simulink model "DTC_step625_20261016_164342_084"  (R2025b)
settings: Solver=FixedStepDiscrete  StartTime=0  StopTime=3.5  FixedStep=6.2500000000000005e-07  MaxStep=1e-3  RelTol=1e-3  EnableMultiTasking=on
model workspace (MAT data in the model file):
  F = 0.0106
  H = 0.2734
  IphasePeak = 243.46443504
  J_kgm2 = 2.52388816871
  Ki_wr = 3134.2
  Kp_wr = 65.47
  Llr_H = 0.000328787586604
  Llr_pu = 0.067199338843
  Lls_H = 0.000328787586604
  Lm_H = 0.0132934166218
  Lm_pu = 2.7169785124
  Pn = 164000
  Rr_pu = 0.0112002512397
  Rrr = 0.020659
  Rss = 0.025639
  Tbase = 870.047022236
  Ts = 6.25e-07
  Tsc = 5e-05
  Vdc = 750
  Vn = 550
  VphasePeak = 449.07311951
  Xlr = 0.12395
  Xls = 0.12395
  Xm = 5.0115
  Zbase = 1.84451219512
  fn = 60
  fswFOC = 5000
  imRef_pu = 0.36805591043
  omegaBase = 188.495559215
  p = 2
  psin = 1.19120344633
  rpmBase = 1800
undefined symbols (not defined in the file): ee
libraries: nesl_utility x12, ee_lib x10, fl_lib x5, eeAsmDirectTorqueControl x1, slpidlib x1
Description:
  | Asynchronous Machine Direct Torque Control
settings Model: Creator=The MathWorks, Inc.  LastModifiedBy=Ulterior Engineering
settings SolverCC: AlgebraicLoopSolver=TrustRegion  AutoInsertRateTranBlk=on  MaxZcPerStep=1.0
settings DataIOCC: MaxDataPoints=510000  SaveOperatingPoint=on  SaveFormat=StructureWithTime  SaveOutput=off  SignalLogging=off  SignalLoggingName=logsout_InductionMachineDTC
settings OptimizationCC: ReuseModelBlockBuffer=off  ExpressionDepthLimit=2147483647.0  LifeSpan=inf
settings DebuggingCC: AlgebraicLoopMsg=error  SolverPrmCheckMsg=warning  MultiTaskRateTransMsg=warning  UnconnectedInputMsg=warning  UnconnectedOutputMsg=warning  UnconnectedLineMsg=warning  StateNameClashWarn=warning  SFUnexpectedBacktrackingDiag=warning  SFNoUnconditionalDefaultTransitionDiag=warning  SFExecutionAtInitializationDiag=none  ArithmeticOperatorsInVariantConditions=warning
settings HardwareCC: ProdBitPerPointer=32.0  ProdBitPerSizeT=32.0  ProdBitPerPtrDiffT=32.0  ProdLargestAtomicFloat=None  ProdIntDivRoundTo=Undefined  ProdEndianess=Unspecified  ProdWordSize=32.0  ProdHWDeviceType=32-bit Generic
settings ModelReferenceCC: EnableRefExpFcnMdlSchedulingChecks=on  PropagateSignalLabelsOutOfModel=off
settings SFSimCC: SimUseLocalCustomCode=off  CustomCodeUndefinedFunction=UseInterfaceOnly
settings RTWCC: RTWUseLocalCustomCode=off  GPUComputeCapability=3.5  DLArmComputeVersion=19.05
settings CodeAppCC: StateflowObjectComments=on
settings GRTTargetCC: TargetLangStandard=C89/C90 (ANSI)
settings ConfigComp: CovMetricSettings=dw  CovSaveCumulativeToWorkspaceVar=on  CovSaveSingleToWorkspaceVar=on  CovExternalEMLEnable=off  CovSFcnEnable=off
settings SimscapeCC: SimscapeLogSimulationStatistics=on  SimscapeLogName=simlog_InductionMachineDTC  SimscapeLogDecimation=5.0  SimscapeLogDataHistory=510000.0

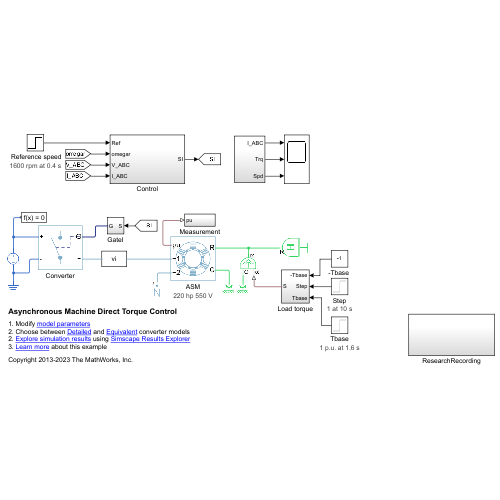
[thumbnail: Simulink's stored preview of the top-level diagram]
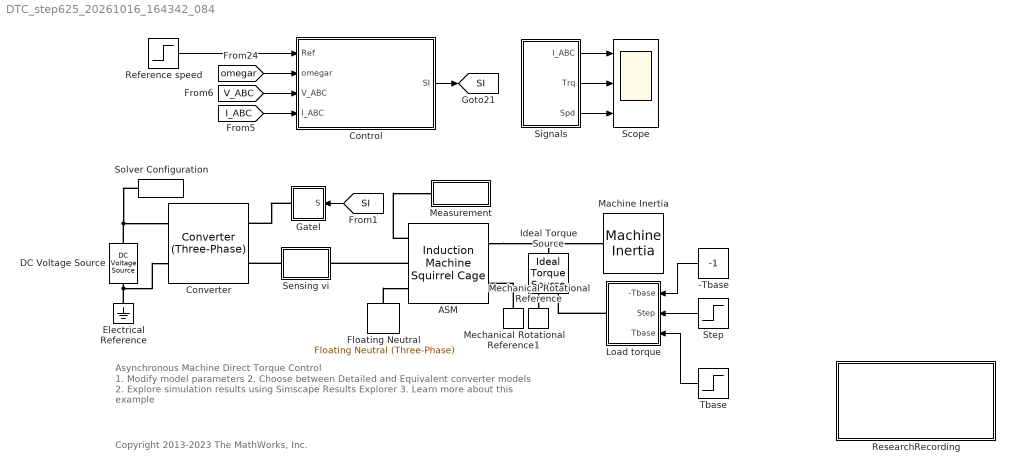
== system DTC_step625_20261016_164342_084 ==
  note: Asynchronous Machine Direct Torque Control
  note: 1. Modify model parameters
      | 2. Choose between Detailed and Equivalent converter models
      | 2. Explore simulation results using Simscape Results Explorer
      | 3. Learn more about this example
  note: Copyright 2013-2023 The MathWorks, Inc.
  " Reference speed" : Step  Time=0.4  After=1600  SampleTime=Tsc
      settings: AttributesFormatString=%<After> rpm at %<Time> s
  "-Tbase " : Constant  Value=-1  SampleTime=Ts
  ASM : ee_lib/Electromechanical/Asynchronous/Induction Machine Squirrel Cage  port_option=ee.enum.threePhasePort.composite  SRated=Pn V*A  VRated=Vn V  FRated=fn Hz  nPolePairs=p  param_unit=ee.enum.unit.si  squirrel_cage=ee.enum.squirrelcage.Single  zero_sequence=ee.enum.park.zerosequence.include  initialization_option=ee.enum.asm.initialization.fluxvariables  Rs=Rss Ohm  Xls=Xls Ohm  pu_Rs=0.0258  pu_Lls=0.0413  Rrd=0.020659 Ohm  Xlrd=Xlr Ohm  pu_Rrd=0.0145  pu_Llrd=0.0424  Rrd1=0.28 Ohm  Xlrd1=0.82 Ohm  Rrd2=0.28 Ohm  Xlrd2=0.82 Ohm  pu_Rrd1=0.0290  pu_Llrd1=0.0848  pu_Rrd2=0.0290  pu_Llrd2=0.0848  Xm=Xm Ohm  pu_Lm=1.7562  X0=Xls Ohm  pu_L0=0.0413  saturation_option=0  saturation_i=[0, 4, 9, 18, 25, 34, 50, 68, 95, 120] A  saturation_v=[0, 88, 154, 198, 220, 242, 264, 286, 308, 330] V  pu_saturation_i=[0, .176, .396, .792, 1.1, 1.496, 2.2, 2.992, 4.18, 5.28]  pu_saturation_v=[0, .4, .7, .9, 1, 1.1, 1.2, 1.3, 1.4, 1.4864]  connection_option=int32(ee.enum.Connection.delta)  angular_position_specify=off  angular_position_priority=None  angular_position=0 deg  angular_position_nominal_specify=off  angular_position_nominal_value=1  angular_position_nominal_unit=deg  pu_psids_specify=off  pu_psids_priority=None  pu_psids=0  pu_psids_nominal_specify=off  pu_psids_nominal_value=1  pu_psids_nominal_unit=1  pu_psiqs_specify=off  pu_psiqs_priority=None  pu_psiqs=0  pu_psiqs_nominal_specify=off  pu_psiqs_nominal_value=1  pu_psiqs_nominal_unit=1  pu_psi0s_specify=off  pu_psi0s_priority=None  pu_psi0s=0  pu_psi0s_nominal_specify=off  pu_psi0s_nominal_value=1  pu_psi0s_nominal_unit=1  pu_psidr_specify=off  pu_psidr_priority=None  pu_psidr=0  pu_psidr_nominal_specify=off  pu_psidr_nominal_value=1  pu_psidr_nominal_unit=1  pu_psiqr_specify=off  pu_psiqr_priority=None  pu_psiqr=0  pu_psiqr_nominal_specify=off  pu_psiqr_nominal_value=1  pu_psiqr_nominal_unit=1  pu_psidr1_specify=off  pu_psidr1_priority=None  pu_psidr1=0  pu_psidr1_nominal_specify=off  pu_psidr1_nominal_value=1  pu_psidr1_nominal_unit=1  pu_psiqr1_specify=off  pu_psiqr1_priority=None  pu_psiqr1=0  pu_psiqr1_nominal_specify=off  pu_psiqr1_nominal_value=1  pu_psiqr1_nominal_unit=1  pu_psidr2_specify=off  pu_psidr2_priority=None  pu_psidr2=0  pu_psidr2_nominal_specify=off  pu_psidr2_nominal_value=1  pu_psidr2_nominal_unit=1  pu_psiqr2_specify=off  pu_psiqr2_priority=None  pu_psiqr2=0  pu_psiqr2_nominal_specify=off  pu_psiqr2_nominal_value=1  pu_psiqr2_nominal_unit=1  psids_specify=off  psids_priority=None  psids=0 Wb  psids_nominal_specify=off  psids_nominal_value=1  psids_nominal_unit=Wb  psiqs_specify=off  psiqs_priority=None  psiqs=0 Wb  psiqs_nominal_specify=off  psiqs_nominal_value=1  psiqs_nominal_unit=Wb  psi0s_specify=off  psi0s_priority=None  psi0s=0 Wb  psi0s_nominal_specify=off  psi0s_nominal_value=1  psi0s_nominal_unit=Wb  psidr_specify=off  psidr_priority=None  psidr=0 Wb  psidr_nominal_specify=off  psidr_nominal_value=1  psidr_nominal_unit=Wb  psiqr_specify=off  psiqr_priority=None  psiqr=0 Wb  psiqr_nominal_specify=off  psiqr_nominal_value=1  psiqr_nominal_unit=Wb  psidr1_specify=off  psidr1_priority=None  psidr1=0 Wb  psidr1_nominal_specify=off  psidr1_nominal_value=1  psidr1_nominal_unit=Wb  psiqr1_specify=off  psiqr1_priority=None  psiqr1=0 Wb  psiqr1_nominal_specify=off  psiqr1_nominal_value=1  psiqr1_nominal_unit=Wb  psidr2_specify=off  psidr2_priority=None  psidr2=0 Wb  psidr2_nominal_specify=off  psidr2_nominal_value=1  psidr2_nominal_unit=Wb  psiqr2_specify=off  psiqr2_priority=None  psiqr2=0 Wb  psiqr2_nominal_specify=off  psiqr2_nominal_value=1  psiqr2_nominal_unit=Wb  slip_specify=off  slip_priority=None  slip=0  slip_nominal_specify=off  slip_nominal_value=1  slip_nominal_unit=1  real_power_generated_specify=off  real_power_generated_priority=None  real_power_generated=0 W  real_power_generated_nominal_specify=off  real_power_generated_nominal_value=1  real_power_generated_nominal_unit=W  mechanical_power_consumed_specify=off  mechanical_power_consumed_priority=None  mechanical_power_consumed=0 W  mechanical_power_consumed_nominal_specify=off  mechanical_power_consumed_nominal_value=1  mechanical_power_consumed_nominal_unit=W  Tmeas=298.15 K  alpha=3.93e-3 1/K  alpha_cage=4.4e-3 1/K  stator_thermal_mass=100 J/K  rotor_thermal_mass=200 J/K  temperatureA_specify=off  temperatureA_priority=High  temperatureA=25 degC  temperatureA_nominal_specify=off  temperatureA_nominal_value=1  temperatureA_nominal_unit=degC  temperatureB_specify=off  temperatureB_priority=High  temperatureB=25 degC  temperatureB_nominal_specify=off  temperatureB_nominal_value=1  temperatureB_nominal_unit=degC  temperatureC_specify=off  temperatureC_priority=High  temperatureC=25 degC  temperatureC_nominal_specify=off  temperatureC_nominal_value=1  temperatureC_nominal_unit=degC  temperatureR_specify=off  temperatureR_priority=High  temperatureR=25 degC  temperatureR_nominal_specify=off  temperatureR_nominal_value=1  temperatureR_nominal_unit=degC
      settings: AttributesFormatString=220 hp 550 V  InternalSimscapePortConfiguration="{\"Bottom\":[],\"Left\":[{\"id\":\"R\",\"label\":\"R\",\"type\":\"foundation.mechanical.rotational.rotational\"},{\"id\":\"C\",\"label\":\"C\",\"type\":\"foundation.mechanical.rotational.rotational\"}],\"Right\":[{\"id\":\"pu_output\",\"label\":\"pu\",\"type\":\"output\"},{\"id\":\"N1\",\"label\":\"~1\",\"type\":\"foundation.electrical.three_phase\"},{\"id\":\"N2\",\"label\":\"~2\",\"type\":\"foundation.electrical.three_phase\"}],\"Top\":[]}"
  Control : Subsystem
  Converter : ee_lib/Semiconductors & Converters/Converters/Converter (Three-Phase)  port_option=ee.enum.threePhasePort.composite  fidelity_option=ee.enum.converters.fidelity.detailed  device_type=3  showThermalPort=false  K=0  Vth=0.5 V  Vgt=1 V  Vgt_off=-1 V  Ih=1 A  Vf=0.8 V  Ron=0.001 Ohm  Rds=0.001 Ohm  Goff=1e-5 1/Ohm  Eon_scalar=22.86e-3 J  Eoff_scalar=17.14e-3 J  Eoff_natural_commutation=10e-3 J  Voff=300 V  Iout_scalar=600 A  onCurrentMeasDelay=0 s  useCurrentFromPreviousCycle=false  useVoltageFromPreviousCycle=false  diode_param=2  diode_Vf=0.8 V  diode_Ron=0.001 Ohm  diode_Goff=1e-5 1/Ohm  diode_C=50 nF  diode_iRM=-235 A  diode_iF=300 A  diode_idot=-50 A/us  diode_trr_param=1  diode_trr_factor=3  diode_trr=15 us  diode_Qrr=1.5e+3 s*uA  diode_rec_loss_model=ee.enum.diode.reverseRecoveryModel.fixed  diode_ErecVal=0 J  diode_scaleWithIandV=false  diode_ErecMat=zeros(2, 3) J  diode_TjrecVec=[298.15, 398.15] K  diode_IfrecVec=[.1, 1, 10] A  diode_IrecVal=10 A  diode_VrecVal=10 V  diode_tFilter=1 / 1000 / 100 s  thermal_network_parameterization=ee.enum.thermalNetworkTopology.external  Rth=[.08, .5] K/W  Rth_Cauer=[.08, .1, .5] K/W  Rth_Foster=[.08, .14, .22, .16] K/W  thermal_mass_parameterization=ee.enum.thermalNetwork.timeconstant  thermal_mass=[.01, .5] J/K  thermal_mass_Cauer=[.01, .1, .5] J/K  thermal_mass_Foster=[.001, .005, .05, .5] J/K  thermal_time_constant=[.001, .2] s  thermal_time_constant_Cauer=[.001, .1, .2] s  thermal_time_constant_Foster=[7e-05, .0007, .01, .08] s  thermal_mass_initial_temperatures=[25, 25] degC  thermal_mass_initial_temperatures_Cauer=[25, 25, 25] degC  junction_thermal_mass=0.01 J/K  Tvec_initial_Foster=[25, 25, 25, 25] degC  snubber_type=0  Cs=1e-7 F  Rs=0.1 Ohm  Vce_loss=[0, 150, 300] V
  DC Voltage Source : fl_lib/Electrical/Electrical Sources/DC Voltage Source  v0=750 V
  Electrical Reference : fl_lib/Electrical/Electrical Elements/Electrical Reference
  Floating Neutral : ee_lib/Connectors & References/Floating Neutral (Three-Phase)  G_parasitic=1e-12 1/Ohm
      settings: InternalSimscapePortConfiguration="{\"Bottom\":[],\"Left\":[{\"id\":\"N\",\"label\":\"~\",\"type\":\"foundation.electrical.three_phase\"}],\"Right\":[],\"Top\":[]}"
  GateI : Subsystem
  Ideal Torque Source : fl_lib/Mechanical/Mechanical Sources/Ideal Torque Source
  Load torque : Subsystem
  Machine Inertia : ee_lib/Electromechanical/Mechanical/Machine Inertia  SRated=Pn V*A  FRated=fn Hz  nPolePairs=p  inertia_option=2  J=27548 kg*m^2  H=H s*W/V/A  damper_option=2  D=39.0509 N*m/(rad/s)  pu_D=F  initialization_option=2  fMechanical0=60 Hz  fElectrical0=0 Hz
      settings: InternalSimscapePortConfiguration="{\"Bottom\":[],\"Left\":[{\"id\":\"R\",\"label\":\"R\",\"type\":\"foundation.mechanical.rotational.rotational\"}],\"Right\":[],\"Top\":[]}"
  Measurement : Subsystem
  Mechanical Rotational Reference : fl_lib/Mechanical/Rotational Elements/Mechanical Rotational Reference
  Mechanical Rotational Reference1 : fl_lib/Mechanical/Rotational Elements/Mechanical Rotational Reference
  ResearchRecording : Subsystem
  Scope : Scope  NumInputPorts=3
      settings: ActiveDisplayYMinimum=-2097.68895  ActiveDisplayYMaximum=2224.93237
  Sensing vi : Subsystem
      mask Display: disp('vi')
  Signals : Subsystem
  Solver Configuration : nesl_utility/Solver Configuration  PhysicalDomain=network_engine_domain  SubClassName=solver  LeftPortType=input  RightPortType=generic  Tones=[]  Harmonics=[]  SimulateNoise=off  Profile=off  UseLocalSampling=off  EnableSwitchedLinearOptims=on  FrequencyDomain=off  UseCCode=off  RelTol=0.001  AbsTol=1e-06  MinStep=1e-09  ToWorkspace=off  RevertToSquareIcSolve=off  NumHomotopyIterations=100  PhasorMode=off  PhasorModeNumHarmonics=1  ConsistencySolver=NEWTON_FTOL  IndexReductionMethod=DerivativeReplacement  DoDC=off  ResidualTolerance=1e-09  ConsistencyTolSource=GLOBAL  ConsistencyAbsTol=0.001  ConsistencyRelTol=0.001  ConsistencyTolFactor=0.001  UseLocalSolver=on  LocalSolverChoice=NE_BACKWARD_EULER_ADVANCER  ResolveIndetEquations=on  FunctionEvalNumThread=1  LocalSolverSampleTime=6.2500000000000005e-07  DoFixedCost=on  MaxNonlinIter=10  MaxModeIter=4  ComputeImpulses=off  ImpulseIterations=2  LinearAlgebra=auto  LinearAlgebraNumThread=0  EquationFormulation=NE_TIME_EF  DelaysMemoryBudget=1024  AutomaticFiltering=on  FilteringTimeConstant=0.001  PartitionStorageMethod=AS_NEEDED  PartitionMemoryBudget=1024  PartitionMethod=ROBUST  MultibodyUseLocalSolver=off  MultibodyLocalSolverChoice=ODE1  MultibodyLocalSolverSampleTime=0.001
  Step : Step  Time=10  SampleTime=Ts
      settings: AttributesFormatString=%<After> at %<Time> s
  Tbase : Step  Time=1.6  SampleTime=Ts
      settings: AttributesFormatString=%<After> p.u. at %<Time> s
  tag scope: SI=global
  wires:
  [SI] -> GateI/1(S)
  Signals/1(I_ABC) -> Scope/1
  Signals/2(Trq) -> Scope/2
  Signals/3(Spd) -> Scope/3
  [omegar] -> Control/2(omegar)
  [V_ABC] -> Control/3(V_ABC)
  [I_ABC] -> Control/4(I_ABC)
  Control/1(SI) -> [SI]
  "-Tbase "/1 -> Load torque/1(-Tbase)
  Step/1 -> Load torque/2(Step)
  Tbase/1 -> Load torque/3(Tbase)
  " Reference speed"/1 -> Control/1(Ref)
  connections:
  DC Voltage Source/LConn1 -- Solver Configuration/RConn1 -- Converter/RConn1
  Electrical Reference/LConn1 -- Converter/RConn2 -- DC Voltage Source/RConn1
  Sensing vi/LConn1 -- Converter/LConn2
  ASM/RConn2 -- Sensing vi/RConn1
  ASM/LConn1 -- Ideal Torque Source/LConn1 -- Machine Inertia/LConn1
  Ideal Torque Source/RConn2 -- Mechanical Rotational Reference/LConn1
  GateI/RConn1 -- Converter/LConn1
  Floating Neutral/LConn1 -- ASM/RConn3
  ASM/RConn1 -- Measurement/RConn1
  Mechanical Rotational Reference1/LConn1 -- ASM/LConn2
  Load torque/RConn1 -- Ideal Torque Source/RConn1

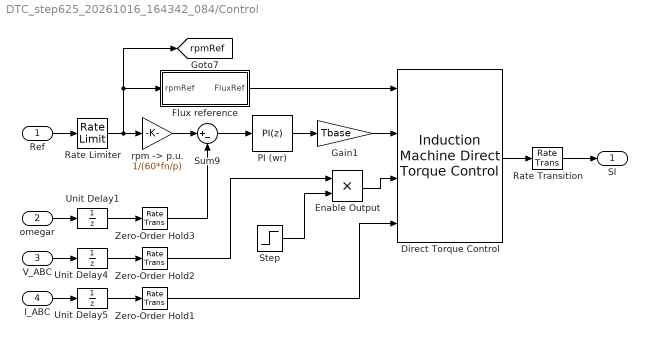
== system DTC_step625_20261016_164342_084/Control ==
  Ref : Inport
  omegar : Inport  Port=2
  V_ABC : Inport  Port=3
  I_ABC : Inport  Port=4
  " Direct Torque Control" : eeAsmDirectTorqueControl/Induction Machine Direct Torque Control  Rs=Rss  p=p  FluxHystBand=.2  THystBand=100  Ts=Tsc
  Enable Output : Product
  Flux reference : Subsystem
  Gain1 : Gain  Gain=Tbase
  PI (wr) : slpidlib/PID Controller  Controller=PI  Form=Parallel  TimeDomain=Discrete-time  UseExternalTs=off  SampleTime=Tsc  IntegratorMethod=Forward Euler  FilterMethod=Forward Euler  ControllerParametersSource=internal  P=Kp_wr  I=Ki_wr  UseKiTs=off  D=0  UseExternalDerivativeSource=off  N=100  UseFilter=on  TunerSelectOption=Transfer Function Based (PID Tuner App)  InitialConditionSource=internal  InitialConditionForIntegrator=0  InitialConditionForFilter=0  DifferentiatorICPrevScaledInput=0  ExternalReset=none  TrackingMode=off  Kt=1  LimitOutput=on  SatLimitsSource=internal  UpperSaturationLimit=2  LowerSaturationLimit=-2  LinearizeAsGain=on  AntiWindupMode=back-calculation  Kb=1000  LimitIntegrator=off  UpperIntegratorSaturationLimit=inf  LowerIntegratorSaturationLimit=-inf  POutMin=[]  POutMax=[]  IOutMin=[]  IOutMax=[]  DOutMin=[]  DOutMax=[]  NOutMin=[]  NOutMax=[]  SumOutMin=[]  SumOutMax=[]  SaturationOutMin=[]  SaturationOutMax=[]  PParamMin=[]  PParamMax=[]  IParamMin=[]  IParamMax=[]  DParamMin=[]  DParamMax=[]  NParamMin=[]  NParamMax=[]  KbParamMin=[]  KbParamMax=[]  KtParamMin=[]  KtParamMax=[]  KbOutMin=[]  KbOutMax=[]  KtOutMin=[]  KtOutMax=[]  IntegratorOutMin=[]  IntegratorOutMax=[]  FilterOutMin=[]  FilterOutMax=[]  SumI1OutMin=[]  SumI1OutMax=[]  SumI2OutMin=[]  SumI2OutMax=[]  SumI3OutMin=[]  SumI3OutMax=[]  SumI4OutMin=[]  SumI4OutMax=[]  SumDOutMin=[]  SumDOutMax=[]  DifferentiatorOutMin=[]  DifferentiatorOutMax=[]  FilterDiffOutCoefMin=[]  FilterDiffOutCoefMax=[]  ReciprocalOutMin=[]  ReciprocalOutMax=[]  SumDenOutMin=[]  SumDenOutMax=[]  SumNumOutMin=[]  SumNumOutMax=[]  DivideOutMin=[]  DivideOutMax=[]  UdiffTsProdOutMin=[]  UdiffTsProdOutMax=[]  NTsProdOutMin=[]  NTsProdOutMax=[]  UintegralTsProdOutMin=[]  UintegralTsProdOutMax=[]  UngainTsProdOutMin=[]  UngainTsProdOutMax=[]  ClampingZeroOutDataTypeStr=Inherit: Inherit via back propagation  ClampingZeroOutMin=[]  ClampingZeroOutMax=[]  FilterDenConstantOutDataTypeStr=Inherit: Inherit via back propagation  FilterDenConstantOutMin=[]  FilterDenConstantOutMax=[]  PCopyOutDataTypeStr=Inherit: Inherit via back propagation  PCopyOutMin=[]  PCopyOutMax=[]  NCopyOutDataTypeStr=Inherit: Inherit via back propagation  NCopyOutMin=[]  NCopyOutMax=[]  IntegratorContinuousStateAttributes=''  IntegratorStateMustResolveToSignalObject=off  IntegratorRTWStateStorageClass=Auto  FilterContinuousStateAttributes=''  FilterStateMustResolveToSignalObject=off  FilterRTWStateStorageClass=Auto  ParallelPVariant=InternalParameters  IdealPVariant=Disabled  IVariant=InternalParameters  DVariant=Disabled  IntegratorVariant=Discrete  SatVariant=Enabled  AWVariant=BackCalculation  PCopyVariant=Disabled  TRVariant=Disabled  FdbkBlocksVariant=Forward  IdealPFdbkVariant=Disabled  SatFdbkVariant=Disabled  DerivativeFilterVariant=Disabled  NVariant=Disabled  NCopyVariant=Disabled_SignalSpec  FilterICVariant=Disabled  IntegratorICVariant=InternalICs  ExternalResetVariant=Disabled  TRSumVariant=Passthrough  SumFdbkVariant=Disabled  SumVariant=Sum_PI  TsampFilterVariant=InternalTs  TsampNgainVariant=Passthrough  TsampIntegralVariant=Disabled_SignalSpec  ExternalSaturationOutDataTypeStr=Inherit: Same as second input  DerivativeSourceVariant=Disabled  PreIntVariant=InternalPreInt
  Rate Limiter : RateLimiter  RisingSlewLimit=2000  FallingSlewLimit=-2000  SampleTimeMode=inherited
      settings: AttributesFormatString=%<RisingSlewLimit> rpm/s
  Rate Transition : RateTransition
  Step : Step  Time=0.1  SampleTime=Tsc
      settings: AttributesFormatString=%<After> at %<Time> s
  Sum9 : Sum  Inputs=|+-
  Unit Delay1 : UnitDelay  SampleTime=5e-6  HasFrameUpgradeWarning=on
  Unit Delay4 : UnitDelay  SampleTime=5e-6  HasFrameUpgradeWarning=on
  Unit Delay5 : UnitDelay  SampleTime=5e-6  HasFrameUpgradeWarning=on
  Zero-Order Hold1 : RateTransition  OutPortSampleTime=5e-05
  Zero-Order Hold2 : RateTransition  OutPortSampleTime=5e-05
  Zero-Order Hold3 : RateTransition  OutPortSampleTime=5e-05
  "rpm -> p.u." : Gain  Gain=1/(60*fn/p)
  SI : Outport  VectorParamsAs1DForOutWhenUnconnected=off
  tag scope: rpmRef=global
  wires:
  Gain1/1 -> " Direct Torque Control"/2
  Step/1 -> Enable Output/2
  Sum9/1 -> PI (wr)/1
  "rpm -> p.u."/1 -> Sum9/1
  Zero-Order Hold1/1 -> " Direct Torque Control"/4
  Unit Delay1/1 -> Zero-Order Hold3/1
  Flux reference/1(FluxRef) -> " Direct Torque Control"/1
  PI (wr)/1 -> Gain1/1
  Zero-Order Hold3/1 -> Sum9/2
  Rate Limiter/1 -> [rpmRef], Flux reference/1(rpmRef), "rpm -> p.u."/1
  V_ABC/1 -> Unit Delay4/1
  omegar/1 -> Unit Delay1/1
  Unit Delay5/1 -> Zero-Order Hold1/1
  Unit Delay4/1 -> Zero-Order Hold2/1
  " Direct Torque Control"/1 -> Rate Transition/1
  I_ABC/1 -> Unit Delay5/1
  Rate Transition/1 -> SI/1
  Enable Output/1 -> " Direct Torque Control"/3
  Zero-Order Hold2/1 -> Enable Output/1
  Ref/1 -> Rate Limiter/1

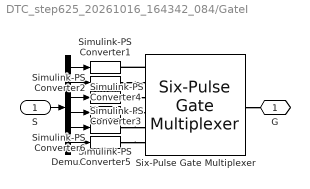
== system DTC_step625_20261016_164342_084/GateI ==
  S : Inport
  Demux : Demux  Outputs=6
  Simulink-PS Converter{1..6} (6 alike) : nesl_utility/Simulink-PS Converter  PhysicalDomain=network_engine_domain  SubClassName=ps_input  LeftPortType=input  RightPortType=output  PseudoPeriodic=off  Frequencies=[]  NoiseDistribution=none  NoiseParameters=[]  Unit=1  AffineConversion=off  FilteringAndDerivatives=zero  SimscapeFilterOrder=1  InputFilterTimeConstant=0.001  UdotUserProvided=1
  Six-Pulse Gate Multiplexer : ee_lib/Semiconductors & Converters/Converters/Six-Pulse Gate Multiplexer  port_option=ee.enum.controlport.ps
  G : PMIOPort  Side=Right
  wires:
  Demux/3 -> Simulink-PS Converter3/1
  Demux/6 -> Simulink-PS Converter6/1
  Demux/5 -> Simulink-PS Converter5/1
  S/1 -> Demux/1
  Demux/2 -> Simulink-PS Converter2/1
  Demux/1 -> Simulink-PS Converter1/1
  Demux/4 -> Simulink-PS Converter4/1
  connections:
  Six-Pulse Gate Multiplexer/RConn1 -- G/RConn1
  Six-Pulse Gate Multiplexer/LConn1 -- Simulink-PS Converter1/RConn1
  Simulink-PS Converter5/RConn1 -- Six-Pulse Gate Multiplexer/LConn5
  Simulink-PS Converter6/RConn1 -- Six-Pulse Gate Multiplexer/LConn6
  Simulink-PS Converter3/RConn1 -- Six-Pulse Gate Multiplexer/LConn3
  Simulink-PS Converter2/RConn1 -- Six-Pulse Gate Multiplexer/LConn2
  Simulink-PS Converter4/RConn1 -- Six-Pulse Gate Multiplexer/LConn4

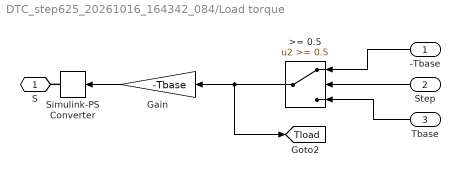
== system DTC_step625_20261016_164342_084/Load torque ==
  -Tbase : Inport
  Step : Inport  Port=2
  Tbase : Inport  Port=3
  ">= 0.5 " : Switch  Threshold=0.5  SaturateOnIntegerOverflow=off  InputSameDT=off
  Gain : Gain  Gain=-Tbase
  Simulink-PS Converter : nesl_utility/Simulink-PS Converter  PhysicalDomain=network_engine_domain  SubClassName=ps_input  LeftPortType=input  RightPortType=output  PseudoPeriodic=off  Frequencies=[]  NoiseDistribution=none  NoiseParameters=[]  Unit=1  AffineConversion=off  FilteringAndDerivatives=zero  SimscapeFilterOrder=1  InputFilterTimeConstant=0.001  UdotUserProvided=1
  S : PMIOPort  Side=Right
  tag scope: Tload=global
  wires:
  Tbase/1 -> ">= 0.5 "/3
  ">= 0.5 "/1 -> Gain/1, [Tload]
  Gain/1 -> Simulink-PS Converter/1
  Step/1 -> ">= 0.5 "/2
  -Tbase/1 -> ">= 0.5 "/1
  connections:
  Simulink-PS Converter/RConn1 -- S/RConn1

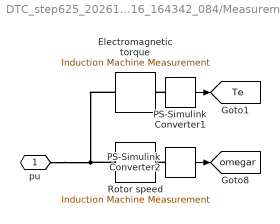
== system DTC_step625_20261016_164342_084/Measurement ==
  Electromagnetic torque : ee_lib/Electromechanical/Asynchronous/Induction Machine Measurement  output_idx=1
      settings: InternalSimscapePortConfiguration="{\"Bottom\":[],\"Left\":[{\"id\":\"pu_input\",\"label\":\"pu\",\"type\":\"input\"}],\"Right\":[{\"id\":\"pu_output\",\"label\":\"o\",\"type\":\"output\"}],\"Top\":[]}"
  PS-Simulink Converter1 : nesl_utility/PS-Simulink Converter  PhysicalDomain=network_engine_domain  SubClassName=ps_output  LeftPortType=input  RightPortType=output  PseudoPeriodic=off  Frequencies=[]  VectorFormat=1-D array  Unit=1  AffineConversion=off
  PS-Simulink Converter2 : nesl_utility/PS-Simulink Converter  PhysicalDomain=network_engine_domain  SubClassName=ps_output  LeftPortType=input  RightPortType=output  PseudoPeriodic=off  Frequencies=[]  VectorFormat=1-D array  Unit=1  AffineConversion=off
  Rotor speed : ee_lib/Electromechanical/Asynchronous/Induction Machine Measurement  output_idx=2
      settings: InternalSimscapePortConfiguration="{\"Bottom\":[],\"Left\":[{\"id\":\"pu_input\",\"label\":\"pu\",\"type\":\"input\"}],\"Right\":[{\"id\":\"pu_output\",\"label\":\"o\",\"type\":\"output\"}],\"Top\":[]}"
  pu : PMIOPort  Side=Right
  tag scope: Te=global, omegar=global
  wires:
  PS-Simulink Converter2/1 -> [omegar]
  PS-Simulink Converter1/1 -> [Te]
  connections:
  PS-Simulink Converter2/LConn1 -- Rotor speed/RConn1
  PS-Simulink Converter1/LConn1 -- Electromagnetic torque/RConn1
  Electromagnetic torque/LConn1 -- pu/RConn1 -- Rotor speed/LConn1

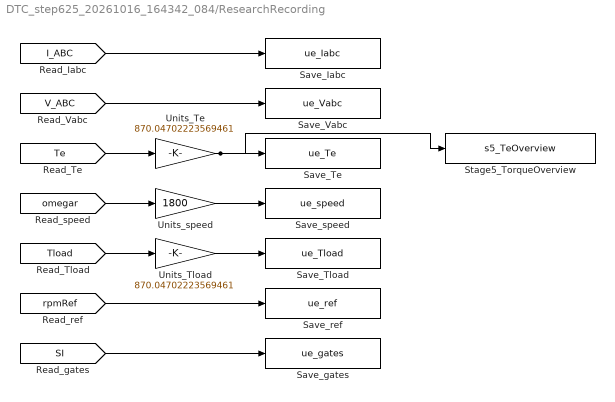
== system DTC_step625_20261016_164342_084/ResearchRecording ==
  Save_Iabc : ToWorkspace  VariableName=ue_Iabc  SaveFormat=Timeseries  SampleTime=-1
      settings: MaxDataPoints=960003
  Save_Te : ToWorkspace  VariableName=ue_Te  SaveFormat=Timeseries  SampleTime=-1
      settings: MaxDataPoints=960003
  Save_Tload : ToWorkspace  VariableName=ue_Tload  SaveFormat=Timeseries  SampleTime=5.0000000000000002e-05
  Save_Vabc : ToWorkspace  VariableName=ue_Vabc  SaveFormat=Timeseries  SampleTime=-1
      settings: MaxDataPoints=960003
  Save_gates : ToWorkspace  VariableName=ue_gates  SaveFormat=Timeseries  SampleTime=-1
      settings: MaxDataPoints=960003
  Save_ref : ToWorkspace  VariableName=ue_ref  SaveFormat=Timeseries  SampleTime=5.0000000000000002e-05
  Save_speed : ToWorkspace  VariableName=ue_speed  SaveFormat=Timeseries  SampleTime=5.0000000000000002e-05
  Stage5_TorqueOverview : ToWorkspace  VariableName=s5_TeOverview  SaveFormat=Timeseries  SampleTime=5.0000000000000002e-05
  Units_Te : Gain  Gain=870.04702223569461
  Units_Tload : Gain  Gain=870.04702223569461
  Units_speed : Gain  Gain=1800
  wires:
  [I_ABC] -> Save_Iabc/1
  [V_ABC] -> Save_Vabc/1
  [Te] -> Units_Te/1
  Units_Te/1 -> Save_Te/1, Stage5_TorqueOverview/1
  [omegar] -> Units_speed/1
  Units_speed/1 -> Save_speed/1
  [Tload] -> Units_Tload/1
  Units_Tload/1 -> Save_Tload/1
  [rpmRef] -> Save_ref/1
  [SI] -> Save_gates/1

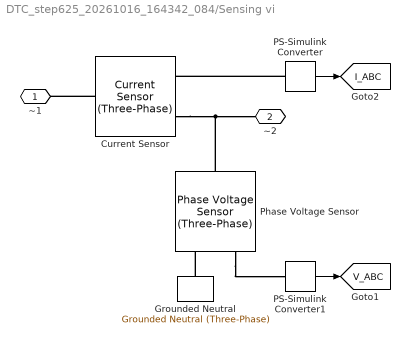
== system DTC_step625_20261016_164342_084/Sensing vi ==
  Current Sensor : ee_lib/Sensors & Transducers/Current Sensor (Three-Phase)
  Grounded Neutral : ee_lib/Connectors & References/Grounded Neutral (Three-Phase)
  PS-Simulink Converter : nesl_utility/PS-Simulink Converter  PhysicalDomain=network_engine_domain  SubClassName=ps_output  LeftPortType=input  RightPortType=output  PseudoPeriodic=off  Frequencies=[]  VectorFormat=1-D array  Unit=A  AffineConversion=off
  PS-Simulink Converter1 : nesl_utility/PS-Simulink Converter  PhysicalDomain=network_engine_domain  SubClassName=ps_output  LeftPortType=input  RightPortType=output  PseudoPeriodic=off  Frequencies=[]  VectorFormat=1-D array  Unit=V  AffineConversion=off
  Phase Voltage Sensor : ee_lib/Sensors & Transducers/Phase Voltage Sensor (Three-Phase)
  ~1 : PMIOPort  Side=Left
  ~2 : PMIOPort  Port=2  Side=Right
  tag scope: I_ABC=global, V_ABC=global
  wires:
  PS-Simulink Converter/1 -> [I_ABC]
  PS-Simulink Converter1/1 -> [V_ABC]
  connections:
  Current Sensor/LConn1 -- ~1/RConn1
  PS-Simulink Converter/LConn1 -- Current Sensor/RConn1
  Current Sensor/RConn2 -- Phase Voltage Sensor/LConn1 -- ~2/RConn1
  Phase Voltage Sensor/RConn1 -- PS-Simulink Converter1/LConn1
  Grounded Neutral/LConn1 -- Phase Voltage Sensor/RConn2

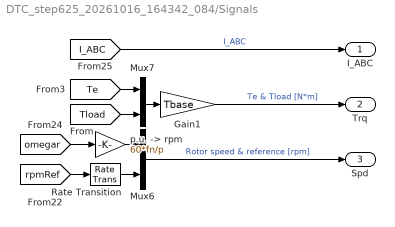
== system DTC_step625_20261016_164342_084/Signals ==
  Gain1 : Gain  Gain=Tbase
  Mux6 : Mux  Inputs=2
  Mux7 : Mux  Inputs=2
  Rate Transition : RateTransition
  "p.u. -> rpm" : Gain  Gain=60*fn/p
  I_ABC : Outport  VectorParamsAs1DForOutWhenUnconnected=off
  Trq : Outport  Port=2  VectorParamsAs1DForOutWhenUnconnected=off
  Spd : Outport  Port=3  VectorParamsAs1DForOutWhenUnconnected=off
  wires:
  [omegar] -> "p.u. -> rpm"/1
  Mux6/1 -> Spd/1  "Rotor speed & reference [rpm]"
  "p.u. -> rpm"/1 -> Mux6/1
  [rpmRef] -> Rate Transition/1
  Rate Transition/1 -> Mux6/2
  [Tload] -> Mux7/2
  [I_ABC] -> I_ABC/1  "I_ABC"
  Mux7/1 -> Gain1/1
  [Te] -> Mux7/1
  Gain1/1 -> Trq/1  "Te & Tload [N*m]"

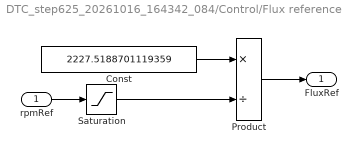
== system DTC_step625_20261016_164342_084/Control/Flux reference ==
  rpmRef : Inport
  Const : Constant  Value=2227.5188701119359
  Product : Product  Inputs=*/
  Saturation : Saturate  UpperLimit=inf  LowerLimit=60*fn/p
  FluxRef : Outport  VectorParamsAs1DForOutWhenUnconnected=off
  wires:
  rpmRef/1 -> Saturation/1
  Product/1 -> FluxRef/1
  Saturation/1 -> Product/2
  Const/1 -> Product/1
